simulink model "pvbattery1"  (R2025a)
settings: Solver=FixedStepAuto  StartTime=0.0  StopTime=86400  FixedStep=1  RelTol=1e-3
libraries: SignalEditorBlockLib x2, simulink x1
settings Model: Creator=Lucas  LastModifiedBy=Lucas

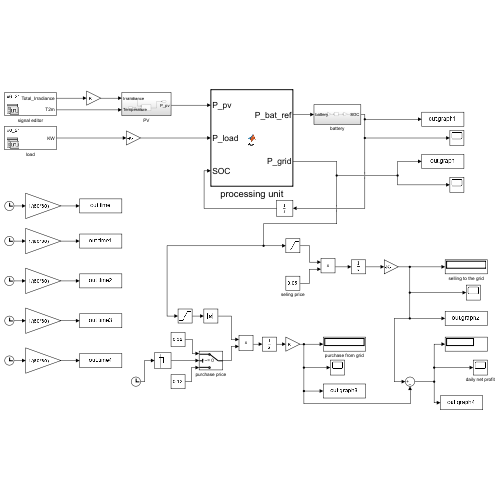
[thumbnail: Simulink's stored preview of the top-level diagram]
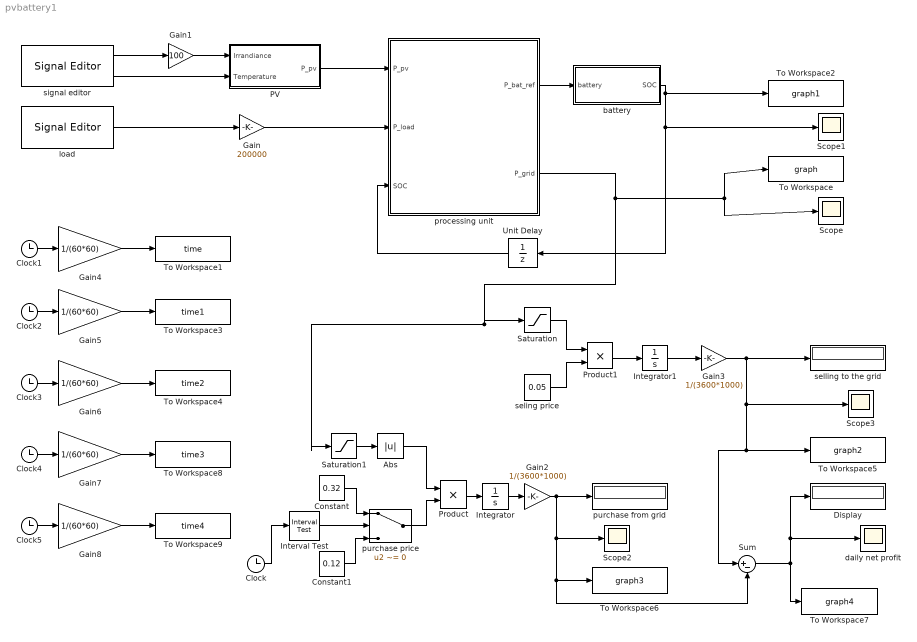
== system pvbattery1 ==
  Abs : Abs  SaturateOnIntegerOverflow=off
  Clock{,1..5} (6 alike) : Clock
  Constant : Constant  Value=0.32
  Constant1 : Constant  Value=0.12
  Display : Display
  Gain : Gain  Gain=200000
  Gain1 : Gain  Gain=100
  Gain2 : Gain  Gain=1/(3600*1000)
  Gain3 : Gain  Gain=1/(3600*1000)
  Gain{4..8} (5 alike) : Gain  Gain=1/(60*60)
  Integrator : Integrator
  Integrator1 : Integrator
  Interval Test : simulink/Logic and Bit Operations/Interval Test  IntervalClosedRight=on  uplimit=75600  IntervalClosedLeft=on  lowlimit=61200  OutDataTypeStr=boolean
  PV : Subsystem
  Product : Product
  Product1 : Product
  Saturation : Saturate  UpperLimit=inf  LowerLimit=0
  Saturation1 : Saturate  UpperLimit=0  LowerLimit=-inf
  Scope{,1..3} (4 alike) : Scope
      Scope settings: ActiveDisplayYMinimum=-176836.75166406349  ActiveDisplayYMaximum=427905.1391701203
      Scope1 settings: ActiveDisplayYMinimum=12.482083570140809  ActiveDisplayYMaximum=87.527942721235178
      Scope2 settings: ActiveDisplayYMinimum=-7.9998267828768217  ActiveDisplayYMaximum=71.998441045891411  DataLoggingVariableName=ScopeData2
      Scope3 settings: ActiveDisplayYMinimum=-13.915719523497188  ActiveDisplayYMaximum=125.24147571147475  DataLoggingVariableName=ScopeData3
  Sum : Sum  Inputs=|+-
  To Workspace : ToWorkspace  VariableName=graph  SampleTime=-1
  To Workspace1 : ToWorkspace  VariableName=time  SampleTime=-1
  To Workspace2 : ToWorkspace  VariableName=graph1  SampleTime=-1
  To Workspace3 : ToWorkspace  VariableName=time1  SampleTime=-1
  To Workspace4 : ToWorkspace  VariableName=time2  SampleTime=-1
  To Workspace5 : ToWorkspace  VariableName=graph2  SampleTime=-1
  To Workspace6 : ToWorkspace  VariableName=graph3  SampleTime=-1
  To Workspace7 : ToWorkspace  VariableName=graph4  SampleTime=-1
  To Workspace8 : ToWorkspace  VariableName=time3  SampleTime=-1
  To Workspace9 : ToWorkspace  VariableName=time4  SampleTime=-1
  Unit Delay : UnitDelay  InitialCondition=50  HasFrameUpgradeWarning=on
  battery : Subsystem
  daily net profit : Scope
      settings: ActiveDisplayYMinimum=-28.372768626877424  ActiveDisplayYMaximum=110.78442660809449  DataLoggingVariableName=ScopeData4
  load : SignalEditorBlockLib/Signal Editor  FileName=C:\Users\Lucas\Desktop\final year project\load_data_waves.mat  ActiveScenario=x6_21  ActiveSignal=KW  IsBus=off  OutputBusObjectStr=Bus: BusObject  SampleTime=0  ZeroCross=off  OutputAfterFinalValue=Setting to zero  Unit=inherit  PreserveSignalName=on  ApplySigPropsToAllScenarios=on  ApplySigPropsToAllSignals=off  SignalPropertySource=Dialog parameters
  processing unit : MATLAB Function  TreatAsAtomicUnit=on
  purchase from grid : Display
  purchase price : Switch  Criteria=u2 ~= 0  Threshold=0.5  SaturateOnIntegerOverflow=off  InputSameDT=off
  seling price : Constant  Value=0.05
  selling to the grid : Display
  signal editor : SignalEditorBlockLib/Signal Editor  FileName=C:\Users\Lucas\Desktop\final year project\data_waves.mat  ActiveScenario=x6_21  ActiveSignal=T2m  IsBus=off  OutputBusObjectStr=Bus: BusObject  SampleTime=0  ZeroCross=off  OutputAfterFinalValue=Setting to zero  Unit=inherit  PreserveSignalName=on  ApplySigPropsToAllScenarios=on  ApplySigPropsToAllSignals=off  SignalPropertySource=Dialog parameters
  wires:
  processing unit/2(P_grid) -> Saturation1/1, Saturation/1, To Workspace/1, Scope/1
  PV/1(P_pv) -> processing unit/1(P_pv)
  processing unit/1(P_bat_ref) -> battery/1(battery)
  battery/1(SOC) -> Unit Delay/1, Scope1/1, To Workspace2/1
  Unit Delay/1 -> processing unit/3(SOC)
  signal editor/1 -> Gain1/1
  signal editor/2 -> PV/2(Temperature)
  load/1 -> Gain/1
  Gain/1 -> processing unit/2(P_load)
  Gain1/1 -> PV/1(Irrandiance)
  Saturation1/1 -> Abs/1
  Integrator/1 -> Gain2/1
  Integrator1/1 -> Gain3/1
  Interval Test/1 -> purchase price/2
  Constant/1 -> purchase price/1
  Constant1/1 -> purchase price/3
  Abs/1 -> Product/1
  Clock/1 -> Interval Test/1
  Product/1 -> Integrator/1
  purchase price/1 -> Product/2
  Gain2/1 -> To Workspace6/1, Sum/2, Scope2/1, purchase from grid/1
  Saturation/1 -> Product1/1
  Product1/1 -> Integrator1/1
  seling price/1 -> Product1/2
  Gain3/1 -> Sum/1, To Workspace5/1, Scope3/1, selling to the grid/1
  Sum/1 -> daily net profit/1, Display/1, To Workspace7/1
  Clock1/1 -> Gain4/1
  Gain4/1 -> To Workspace1/1
  Gain5/1 -> To Workspace3/1
  Clock2/1 -> Gain5/1
  Clock3/1 -> Gain6/1
  Gain6/1 -> To Workspace4/1
  Clock4/1 -> Gain7/1
  Gain7/1 -> To Workspace8/1
  Gain8/1 -> To Workspace9/1
  Clock5/1 -> Gain8/1

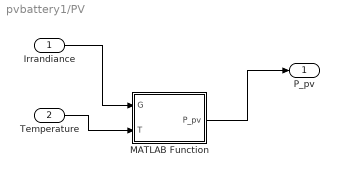
== system pvbattery1/PV ==
  Irrandiance : Inport
  Temperature : Inport  Port=2
  MATLAB Function : MATLAB Function  TreatAsAtomicUnit=on
  P_pv : Outport
  wires:
  Irrandiance/1 -> MATLAB Function/1(G)
  Temperature/1 -> MATLAB Function/2(T)
  MATLAB Function/1(P_pv) -> P_pv/1

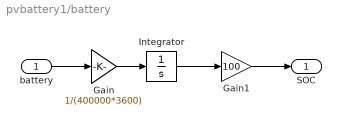
== system pvbattery1/battery ==
  battery : Inport
  Gain : Gain  Gain=1/(400000*3600)
  Gain1 : Gain  Gain=100
  Integrator : Integrator  InitialCondition=0.5  LimitOutput=on  UpperSaturationLimit=1  LowerSaturationLimit=0
  SOC : Outport
  wires:
  battery/1 -> Gain/1
  Gain/1 -> Integrator/1
  Integrator/1 -> Gain1/1
  Gain1/1 -> SOC/1

== matlab function pvbattery1/PV/MATLAB Function ==
  data: G input; P_pv output; T input
function P_pv = fcn(G, T)
    % 按照英国典型的 5kWp 系统设置
    P_nominal = 5000; 
    G_stc = 1000;
    T_stc = 25;
    k = -0.004; % 温度影响系数
    
    % 核心数学模型 (Level 2)
    % 功率与光照成正比，随温度升高略微下降
    P_pv = P_nominal * (G / G_stc) * (1 + k * (T - T_stc));
    
    % 保护逻辑：功率不能小于 0
    if P_pv < 0
        P_pv = 0;
    end
end

== matlab function pvbattery1/processing unit ==
  data: P_pv input; P_bat_ref output; P_load input; SOC input; P_grid output
function [P_bat_ref, P_grid] = fcn(P_pv, P_load, SOC)
    % 定义常量（根据实际毕业设计需求调整）
    SOC_MAX = 80; % 电池电量上限
    SOC_MIN = 20; % 电池电量下限
    
    % 核心逻辑：计算净功率（Net Power）
    % P_net > 0 表示光伏有剩余，P_net < 0 表示光伏不足
    P_net = P_pv - P_load; 

    if P_net > 0 
        % 模式：光伏充足
        if SOC < SOC_MAX
            % 模式：PV -> Bat（优先给电池充电）
            P_bat_ref = P_net; 
            P_grid = 0;
        else
            % 模式：PV -> Grid（电池满了，卖给电网）
            P_bat_ref = 0;
            P_grid = P_net; 
        end
    else
        % 模式：光伏不足
        P_deficit = abs(P_net);
        if SOC > SOC_MIN
            % 模式：Bat -> Load（优先由电池补缺口）
            P_bat_ref = -P_deficit; % 负值代表放电
            P_grid = 0;
        else
            % 模式：Grid -> Load（电池没电了，从电网买电）
            P_bat_ref = 0;
            P_grid = -P_deficit; % 负值代表从电网流入
        end
    end
end
